simulink model "Green_Hydrogen_Model"  (R2026a)
settings: Solver=FixedStepAuto  StopTime=24*3600*365-3600  FixedStep=Ts  AbsTol=1e-3
InitFcn:
  | Ts = 3600;
values from neighbouring files (symbols this model uses):
  zstorage = 5    [initData.mat]
undefined symbols (not defined in the file or in its folder): DiscIntNeverNeededParam
libraries: fl_lib x58, nesl_utility x17, simulink x3, ee_lib x1
CloseFcn:
  | try,close(h1_ee_solar_cell),end
  | clear h1_ee_solar_cell
  | 
  | 
  | clear simlog_ee_solar_cell
  | clear logsout_ee_solar_cell
  | clear I Pmax V_Pmax idx index irradiance irradianceVec legend_info powerMat powerTable temperature temperatureVec vVec voltageTable
Description:
  | Solar Cell Power Curve
settings Model: Creator=The MathWorks, Inc.  LastModifiedBy=aayushi
settings SolverCC: InitialStep=0.1
settings DataIOCC: ExternalInput=[(0:3600:3600*24*365-3600)' irradiance]  LoadExternalInput=on  SaveFormat=StructureWithTime  InspectSignalLogs=on  SignalLoggingName=y  OutputOption=SpecifiedOutputTimes  OutputTimes=[0:0.5:60]
settings DebuggingCC: UnderspecifiedInitializationDetection=Classic
settings HardwareCC: ProdHWDeviceType=32-bit Generic
settings GRTTargetCC: CombineOutputUpdateFcns=off  GRTInterface=on
settings SimscapeCC: SimscapeNormalizeSystem=off  SimscapeNominalValues="[{\"value\":\"1\",\"unit\":\"A\"},{\"value\":\"1\",\"unit\":\"bar\"},{\"value\":\"1\",\"unit\":\"cm^2\"},{\"value\":\"1\",\"unit\":\"cm^3/s\"},{\"value\":\"1\",\"unit\":\"kJ/kg\"},{\"value\":\"1\",\"unit\":\"kW\"},{\"value\":\"1\",\"unit\":\"l\"},{\"value\":\"1\",\"unit\":\"N\"},{\"value\":\"1\",\"unit\":\"N*m\"},{\"value\":\"1\",\"unit\":\"V\"}]"  SimscapeLogType=none  SimscapeLogName=simlog_ee_solar_cell  SimscapeLogLimitData=off

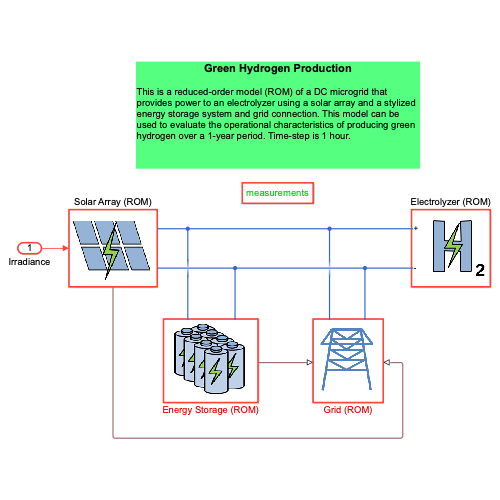
[thumbnail: Simulink's stored preview of the top-level diagram]
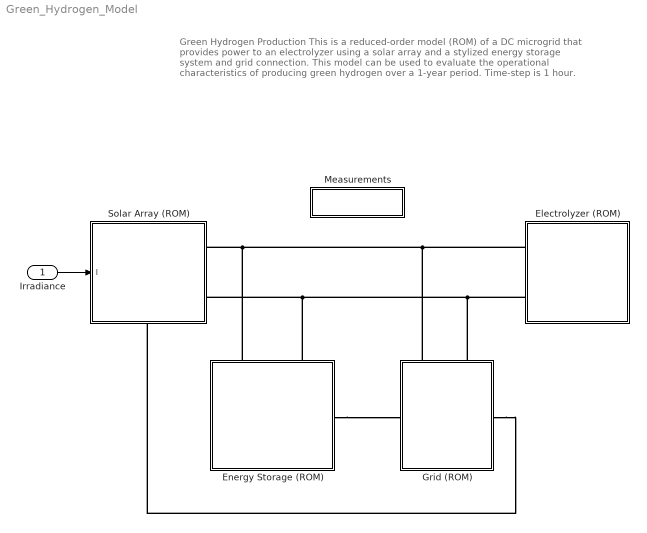
== system Green_Hydrogen_Model ==
  note: Green Hydrogen Production
      |
      | This is a reduced-order model (ROM) of a DC microgrid that provides power to an electrolyzer using a solar array and a stylized energy storage system and grid connection. This model can be used to evaluate the operational characteristics of producing green hydrogen over a 1-year period. Time-step is 1 hour.
  Irradiance : Inport  PortDimensions=1
  Electrolyzer (ROM) : Subsystem
      mask Display: image(imread('green_hydrogen.png'))
  Energy Storage (ROM) : Subsystem
      settings: PortSchema="{\"entries\":[{\"content\":{\"sides\":[{\"content\":{\"connectorIds\":[]},\"type\":\"ConnectorPlacement.EquallySpacedRectSide\",\"uuid\":\"4ce9e896-492d-4425-b4ff-f24d4b5e5863\"},{\"content\":{\"connectorIds\":[\"RConn1\"],\"side\":\"RIGHT\"},\"type\":\"ConnectorPlacement.EquallySpacedRectSide\",\"uuid\":\"930c7228-c80c-44c8-ab76-5d29522f1c4f\"},{\"content\":{\"connectorIds\":[\"LConn1\",\"LConn2\"],\"side\":\"TOP\"},\"type\":\"ConnectorPlacement.EquallySpacedRectSide\",\"uuid\":\"6c2706e8-63c7-47cf-ac96-eabca5dbf54e\"}]},\"type\":\"ConnectorPlacement.EquallySpacedConnector\",\"uuid\":\"1ee3078e-0db2-4038-8bbf-aa4f1eaec25a\"}],\"packageUris\":[\"http://schema.mathworks.com/mf0/Connector/R2020b\"],\"version\":\"1.0\"}"
      mask Display: image(imread('storage.png'))
  Grid (ROM) : Subsystem
      settings: PortSchema="{\"entries\":[{\"content\":{\"sides\":[{\"content\":{\"connectorIds\":[\"LConn1\"]},\"type\":\"ConnectorPlacement.EquallySpacedRectSide\",\"uuid\":\"4ce9e896-492d-4425-b4ff-f24d4b5e5863\"},{\"content\":{\"connectorIds\":[\"RConn1\"],\"side\":\"RIGHT\"},\"type\":\"ConnectorPlacement.EquallySpacedRectSide\",\"uuid\":\"930c7228-c80c-44c8-ab76-5d29522f1c4f\"},{\"content\":{\"connectorIds\":[\"LConn2\",\"LConn3\"],\"side\":\"TOP\"},\"type\":\"ConnectorPlacement.EquallySpacedRectSide\",\"uuid\":\"6c2706e8-63c7-47cf-ac96-eabca5dbf54e\"},{\"content\":{\"connectorIds\":[],\"side\":\"BOTTOM\"},\"type\":\"ConnectorPlacement.EquallySpacedRectSide\",\"uuid\":\"490b5229-98f3-4f3a-9ef5-f546c826e2d2\"}]},\"type\":\"ConnectorPlacement.EquallySpacedConnector\",\"uuid\":\"1ee3078e-0db2-4038-8bbf-aa4f1eaec25a\"}],\"packageUris\":[\"http://schema.mathworks.com/mf0/Connector/R2020b\"],\"version\":\"1.0\"}"
      mask Display: image(imread('grid.png'))
  Measurements : Subsystem
      mask Display: disp('measurements')
  Solar Array (ROM) : Subsystem
      settings: PortSchema="{\"entries\":[{\"content\":{\"sides\":[{\"content\":{\"connectorIds\":[\"In1\"]},\"type\":\"ConnectorPlacement.EquallySpacedRectSide\",\"uuid\":\"a867b3ed-c44d-46d3-b035-bd7f0843dcab\"},{\"content\":{\"connectorIds\":[\"RConn1\",\"RConn2\"],\"side\":\"RIGHT\"},\"type\":\"ConnectorPlacement.EquallySpacedRectSide\",\"uuid\":\"5b118fd7-24ef-441f-9afe-5591aca8fd6c\"},{\"content\":{\"connectorIds\":[],\"side\":\"TOP\"},\"type\":\"ConnectorPlacement.EquallySpacedRectSide\",\"uuid\":\"b5b5fc8b-bb18-419b-a077-b902c124e389\"},{\"content\":{\"connectorIds\":[\"RConn3\"],\"side\":\"BOTTOM\"},\"type\":\"ConnectorPlacement.EquallySpacedRectSide\",\"uuid\":\"62f7ab30-8438-4320-a8c5-25a9418176a3\"}]},\"type\":\"ConnectorPlacement.EquallySpacedConnector\",\"uuid\":\"ded5530a-2615-43e4-9f45-04d72cddf901\"}],\"packageUris\":[\"http://schema.mathworks.com/mf0/Connector/R2020b\"],\"version\":\"1.0\"}"
      mask Display: image(imread('solar.png'))
  wires:
  Irradiance/1 -> Solar Array (ROM)/1(I)
  connections:
  Electrolyzer (ROM)/LConn1 -- Solar Array (ROM)/RConn1 -- Energy Storage (ROM)/LConn1 -- Grid (ROM)/LConn2
  Electrolyzer (ROM)/LConn2 -- Solar Array (ROM)/RConn2 -- Energy Storage (ROM)/LConn2 -- Grid (ROM)/LConn3
  Grid (ROM)/RConn1 -- Solar Array (ROM)/RConn3
  Energy Storage (ROM)/RConn1 -- Grid (ROM)/LConn1

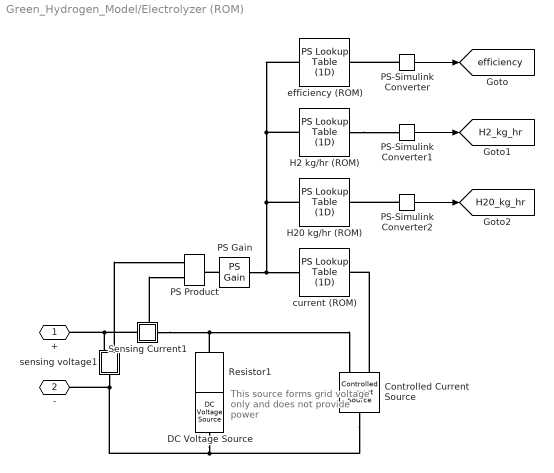
== system Green_Hydrogen_Model/Electrolyzer (ROM) ==
  note: This source forms grid voltage only and does not provide power
  Controlled Current Source : fl_lib/Electrical/Electrical Sources/Controlled Current Source
  DC Voltage Source : fl_lib/Electrical/Electrical Sources/DC Voltage Source  v0=240 V
  H2 kg/hr (ROM) : fl_lib/Physical Signals/Lookup Tables/PS Lookup Table (1D)  x=powerv  f=H2_kg_hr  interp_method=simscape.enum.interpolation.linear  extrap_method=simscape.enum.extrapolation.linear
  H20 kg/hr (ROM) : fl_lib/Physical Signals/Lookup Tables/PS Lookup Table (1D)  x=powerv  f=H20_kg_hr  interp_method=simscape.enum.interpolation.linear  extrap_method=simscape.enum.extrapolation.linear
  PS Gain : fl_lib/Physical Signals/Functions/PS Gain  gain=1 1/V/A
  PS Product : fl_lib/Physical Signals/Functions/PS Product
  PS-Simulink Converter : nesl_utility/PS-Simulink Converter  PhysicalDomain=network_engine_domain  SubClassName=ps_output  LeftPortType=input  RightPortType=output  PseudoPeriodic=off  Frequencies=[]  VectorFormat=1-D array  Unit=inherit  AffineConversion=off
  PS-Simulink Converter1 : nesl_utility/PS-Simulink Converter  PhysicalDomain=network_engine_domain  SubClassName=ps_output  LeftPortType=input  RightPortType=output  PseudoPeriodic=off  Frequencies=[]  VectorFormat=1-D array  Unit=inherit  AffineConversion=off
  PS-Simulink Converter2 : nesl_utility/PS-Simulink Converter  PhysicalDomain=network_engine_domain  SubClassName=ps_output  LeftPortType=input  RightPortType=output  PseudoPeriodic=off  Frequencies=[]  VectorFormat=1-D array  Unit=inherit  AffineConversion=off
  Resistor1 : fl_lib/Electrical/Electrical Elements/Resistor  R=5 Ohm  i_specify=off  i_priority=None  i=0 A  i_nominal_specify=off  i_nominal_value=1  i_nominal_unit=A  v_specify=on  v_priority=None  v=240 V  v_nominal_specify=off  v_nominal_value=1  v_nominal_unit=V
  Sensing Current1 : Subsystem
      settings: PortSchema="{\"entries\":[{\"content\":{\"sides\":[{\"content\":{\"connectorIds\":[\"LConn1\"]},\"type\":\"ConnectorPlacement.EquallySpacedRectSide\",\"uuid\":\"b94629f0-79a7-4e9f-9b19-2ebf3bcf4c67\"},{\"content\":{\"connectorIds\":[\"RConn1\"],\"side\":\"RIGHT\"},\"type\":\"ConnectorPlacement.EquallySpacedRectSide\",\"uuid\":\"77befbbf-81fe-4980-a27e-5f206100ddc5\"},{\"content\":{\"connectorIds\":[\"LConn2\"],\"side\":\"TOP\"},\"type\":\"ConnectorPlacement.EquallySpacedRectSide\",\"uuid\":\"ab227c1c-b66c-46e2-a5f4-7af885246fc6\"}]},\"type\":\"ConnectorPlacement.EquallySpacedConnector\",\"uuid\":\"a3cb571c-cd46-4237-8ad8-7e1205d20cc0\"}],\"packageUris\":[\"http://schema.mathworks.com/mf0/Connector/R2020b\"],\"version\":\"1.0\"}"
      mask Display: disp('i')
  current (ROM) : fl_lib/Physical Signals/Lookup Tables/PS Lookup Table (1D)  x=powerv  f=electrolyzer_current  interp_method=simscape.enum.interpolation.linear  extrap_method=simscape.enum.extrapolation.linear
  efficiency (ROM) : fl_lib/Physical Signals/Lookup Tables/PS Lookup Table (1D)  x=powerv  f=electrolyzer_efficiency  interp_method=simscape.enum.interpolation.linear  extrap_method=simscape.enum.extrapolation.linear
  sensing voltage1 : Subsystem
      mask Display: disp('v')
  + : PMIOPort  Side=Left
  - : PMIOPort  Port=2  Side=Left
  tag scope: H20_kg_hr=global, H2_kg_hr=global, efficiency=global
  wires:
  PS-Simulink Converter/1 -> [efficiency]
  PS-Simulink Converter1/1 -> [H2_kg_hr]
  PS-Simulink Converter2/1 -> [H20_kg_hr]
  connections:
  sensing voltage1/LConn1 -- Sensing Current1/LConn1 -- +/RConn1
  sensing voltage1/RConn1 -- DC Voltage Source/RConn1 -- Controlled Current Source/LConn1 -- -/RConn1
  Sensing Current1/LConn2 -- PS Product/LConn2
  sensing voltage1/LConn2 -- PS Product/LConn1
  PS Gain/LConn1 -- PS Product/RConn1
  Controlled Current Source/RConn1 -- current (ROM)/RConn1
  Sensing Current1/RConn1 -- Resistor1/LConn1 -- Controlled Current Source/RConn2
  DC Voltage Source/LConn1 -- Resistor1/RConn1
  PS-Simulink Converter/LConn1 -- efficiency (ROM)/RConn1
  PS-Simulink Converter2/LConn1 -- H20 kg/hr (ROM)/RConn1
  H2 kg/hr (ROM)/RConn1 -- PS-Simulink Converter1/LConn1
  PS Gain/RConn1 -- current (ROM)/LConn1 -- H20 kg/hr (ROM)/LConn1 -- efficiency (ROM)/LConn1 -- H2 kg/hr (ROM)/LConn1

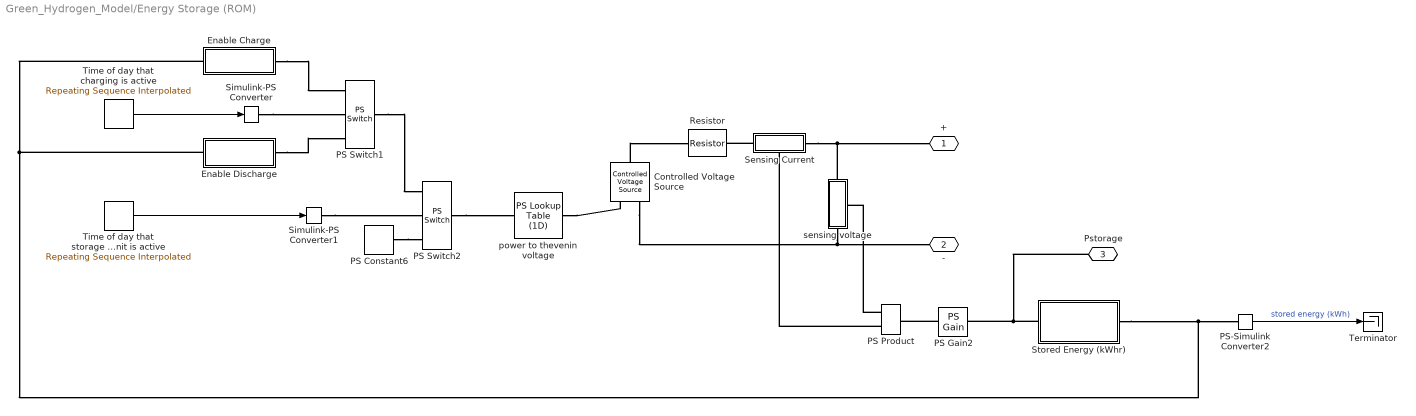
== system Green_Hydrogen_Model/Energy Storage (ROM) ==
  Controlled Voltage Source : fl_lib/Electrical/Electrical Sources/Controlled Voltage Source
  Enable Charge : Subsystem
  Enable Discharge : Subsystem
  PS Constant6 : fl_lib/Physical Signals/Sources/PS Constant  constant=0
  PS Gain2 : fl_lib/Physical Signals/Functions/PS Gain  gain=1 1/V/A
  PS Product : fl_lib/Physical Signals/Functions/PS Product
  PS Switch1 : fl_lib/Physical Signals/Nonlinear Operators/PS Switch  Threshold=0.99  ZeroCross=true
  PS Switch2 : fl_lib/Physical Signals/Nonlinear Operators/PS Switch  Threshold=0.99  ZeroCross=true
  PS-Simulink Converter2 : nesl_utility/PS-Simulink Converter  PhysicalDomain=network_engine_domain  SubClassName=ps_output  LeftPortType=input  RightPortType=output  PseudoPeriodic=off  Frequencies=[]  VectorFormat=1-D array  Unit=inherit  AffineConversion=off
  Resistor : fl_lib/Electrical/Electrical Elements/Resistor  R=zstorage Ohm  i_specify=off  i_priority=None  i=0 A  i_nominal_specify=off  i_nominal_value=1  i_nominal_unit=A  v_specify=off  v_priority=None  v=0 V  v_nominal_specify=off  v_nominal_value=1  v_nominal_unit=V
  Sensing Current : Subsystem
      settings: PortSchema="{\"entries\":[{\"content\":{\"sides\":[{\"content\":{\"connectorIds\":[\"LConn1\"]},\"type\":\"ConnectorPlacement.EquallySpacedRectSide\",\"uuid\":\"c99cf1a8-fc4f-439f-81a5-065ef56794a1\"},{\"content\":{\"connectorIds\":[\"RConn1\"],\"side\":\"RIGHT\"},\"type\":\"ConnectorPlacement.EquallySpacedRectSide\",\"uuid\":\"2fde9b7a-e051-4c9e-865a-56b031831294\"},{\"content\":{\"connectorIds\":[],\"side\":\"TOP\"},\"type\":\"ConnectorPlacement.EquallySpacedRectSide\",\"uuid\":\"fbc77884-485b-4fd8-805c-e7a3dc707aba\"},{\"content\":{\"connectorIds\":[\"RConn2\"],\"side\":\"BOTTOM\"},\"type\":\"ConnectorPlacement.EquallySpacedRectSide\",\"uuid\":\"a7518d99-1e9b-4c67-b1d7-16fc35a4cea4\"}]},\"type\":\"ConnectorPlacement.EquallySpacedConnector\",\"uuid\":\"18321e03-afa8-4af1-9a2f-bf6413052394\"}],\"packageUris\":[\"http://schema.mathworks.com/mf0/Connector/R2020b\"],\"version\":\"1.0\"}"
      mask Display: disp('i')
  Simulink-PS Converter : nesl_utility/Simulink-PS Converter  PhysicalDomain=network_engine_domain  SubClassName=ps_input  LeftPortType=input  RightPortType=output  PseudoPeriodic=off  Frequencies=[]  NoiseDistribution=none  NoiseParameters=[]  Unit=1  AffineConversion=off  FilteringAndDerivatives=provide  SimscapeFilterOrder=1  InputFilterTimeConstant=0.001  UdotUserProvided=0
  Simulink-PS Converter1 : nesl_utility/Simulink-PS Converter  PhysicalDomain=network_engine_domain  SubClassName=ps_input  LeftPortType=input  RightPortType=output  PseudoPeriodic=off  Frequencies=[]  NoiseDistribution=none  NoiseParameters=[]  Unit=1  AffineConversion=off  FilteringAndDerivatives=provide  SimscapeFilterOrder=1  InputFilterTimeConstant=0.001  UdotUserProvided=0
  Stored Energy (kWhr) : Subsystem
  Terminator : Terminator
  Time of day that charging is active : simulink/Sources/Repeating Sequence Interpolated  OutValues=[0 0 1 1 0 0]  TimeValues=[0 8*3600-Ts 8*3600 14*3600-Ts 14*3600 24*3600-Ts]  LookUpMeth=Interpolation-Use End Values  tsamp=Ts  OutMin=[]  OutMax=[]  OutDataTypeStr=double  OutputDataTypeScalingMode=double  OutDataType=fixdt(0,8)  OutScaling=2^-10
  Time of day that storage unit is active : simulink/Sources/Repeating Sequence Interpolated  OutValues=[0 0 1 1 0 0 1 1]  TimeValues=[0 6*3600-Ts 6*3600 12*3600-Ts 12*3600 20*3600-Ts 20*3600 24*3600-Ts]  LookUpMeth=Interpolation-Use End Values  tsamp=Ts  OutMin=[]  OutMax=[]  OutDataTypeStr=double  OutputDataTypeScalingMode=double  OutDataType=fixdt(0,8)  OutScaling=2^-10
  power to thevenin voltage : fl_lib/Physical Signals/Lookup Tables/PS Lookup Table (1D)  x=pstorage  f=vstorage  interp_method=simscape.enum.interpolation.linear  extrap_method=simscape.enum.extrapolation.linear
  sensing voltage : Subsystem
      settings: PortSchema="{\"entries\":[{\"content\":{\"sides\":[{\"content\":{\"connectorIds\":[\"LConn1\"]},\"type\":\"ConnectorPlacement.EquallySpacedRectSide\",\"uuid\":\"174cc4c7-8d7f-48d2-a7e2-2f35130ccdcd\"},{\"content\":{\"connectorIds\":[\"RConn1\"],\"side\":\"RIGHT\"},\"type\":\"ConnectorPlacement.EquallySpacedRectSide\",\"uuid\":\"9e60102e-41cf-47d2-a399-aa8583a1bfd5\"},{\"content\":{\"connectorIds\":[],\"side\":\"TOP\"},\"type\":\"ConnectorPlacement.EquallySpacedRectSide\",\"uuid\":\"1bf2b277-65ab-4966-a80f-8100630a083b\"},{\"content\":{\"connectorIds\":[\"RConn2\"],\"side\":\"BOTTOM\"},\"type\":\"ConnectorPlacement.EquallySpacedRectSide\",\"uuid\":\"735a8926-423a-42f4-bd5d-475d3049eafb\"}]},\"type\":\"ConnectorPlacement.EquallySpacedConnector\",\"uuid\":\"1a25aba2-97b0-44d7-b65c-a2aa0aac9e6e\"}],\"packageUris\":[\"http://schema.mathworks.com/mf0/Connector/R2020b\"],\"version\":\"1.0\"}"
      mask Display: disp('v')
  + : PMIOPort  Side=Left
  - : PMIOPort  Port=2  Side=Left
  Pstorage : PMIOPort  Port=3  Side=Right
  wires:
  PS-Simulink Converter2/1 -> Terminator/1  "stored energy (kWh)"
  Time of day that charging is active/1 -> Simulink-PS Converter/1
  Time of day that storage unit is active/1 -> Simulink-PS Converter1/1
  connections:
  Controlled Voltage Source/LConn1 -- Resistor/RConn1
  Controlled Voltage Source/RConn2 -- sensing voltage/RConn1 -- -/RConn1
  Sensing Current/LConn1 -- Resistor/LConn1
  Sensing Current/RConn1 -- sensing voltage/LConn1 -- +/RConn1
  PS Product/LConn1 -- sensing voltage/RConn2
  PS Product/LConn2 -- Sensing Current/RConn2
  PS Gain2/LConn1 -- PS Product/RConn1
  power to thevenin voltage/RConn1 -- Controlled Voltage Source/RConn1
  PS Switch1/RConn1 -- PS Switch2/LConn1
  PS Constant6/RConn1 -- PS Switch2/LConn3
  PS Switch2/RConn1 -- power to thevenin voltage/LConn1
  Simulink-PS Converter/RConn1 -- PS Switch1/LConn2
  Simulink-PS Converter1/RConn1 -- PS Switch2/LConn2
  Pstorage/RConn1 -- Stored Energy (kWhr)/LConn1 -- PS Gain2/RConn1
  Enable Discharge/RConn1 -- PS Switch1/LConn3
  Stored Energy (kWhr)/RConn1 -- Enable Charge/LConn1 -- Enable Discharge/LConn1 -- PS-Simulink Converter2/LConn1
  Enable Charge/RConn1 -- PS Switch1/LConn1

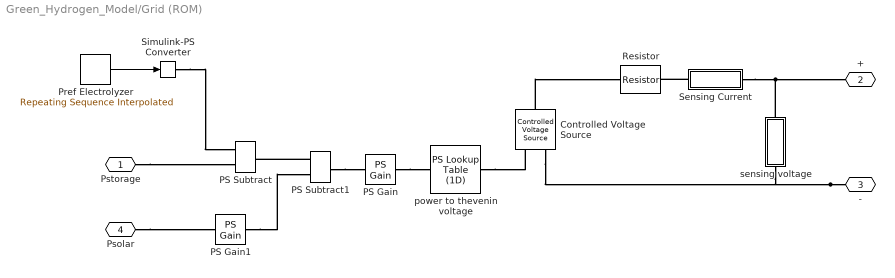
== system Green_Hydrogen_Model/Grid (ROM) ==
  Controlled Voltage Source : fl_lib/Electrical/Electrical Sources/Controlled Voltage Source
  PS Gain : fl_lib/Physical Signals/Functions/PS Gain  gain=1
  PS Gain1 : fl_lib/Physical Signals/Functions/PS Gain  gain=1 1/V/A
  PS Subtract : fl_lib/Physical Signals/Functions/PS Subtract
  PS Subtract1 : fl_lib/Physical Signals/Functions/PS Subtract
  Pref Electrolyzer : simulink/Sources/Repeating Sequence Interpolated  OutValues=[0.01 0.01 1 1 1 1]*150e3  TimeValues=[0 8*3600-Ts 8*3600 20*3600-Ts 20*3600 24*3600-Ts]  LookUpMeth=Interpolation-Use End Values  tsamp=Ts  OutMin=[]  OutMax=[]  OutDataTypeStr=double  OutputDataTypeScalingMode=double  OutDataType=fixdt(0,8)  OutScaling=2^-10
  Resistor : fl_lib/Electrical/Electrical Elements/Resistor  R=zstorage Ohm  i_specify=off  i_priority=None  i=0 A  i_nominal_specify=off  i_nominal_value=1  i_nominal_unit=A  v_specify=off  v_priority=None  v=0 V  v_nominal_specify=off  v_nominal_value=1  v_nominal_unit=V
  Sensing Current : Subsystem
      mask Display: disp('i')
  Simulink-PS Converter : nesl_utility/Simulink-PS Converter  PhysicalDomain=network_engine_domain  SubClassName=ps_input  LeftPortType=input  RightPortType=output  PseudoPeriodic=off  Frequencies=[]  NoiseDistribution=none  NoiseParameters=[]  Unit=1  AffineConversion=off  FilteringAndDerivatives=provide  SimscapeFilterOrder=1  InputFilterTimeConstant=0.001  UdotUserProvided=0
  power to thevenin voltage : fl_lib/Physical Signals/Lookup Tables/PS Lookup Table (1D)  x=pstorage  f=vstorage  interp_method=simscape.enum.interpolation.linear  extrap_method=simscape.enum.extrapolation.linear
  sensing voltage : Subsystem
      mask Display: disp('v')
  Pstorage : PMIOPort  Side=Left
  + : PMIOPort  Port=2  Side=Left
  - : PMIOPort  Port=3  Side=Left
  Psolar : PMIOPort  Port=4  Side=Right
  wires:
  Pref Electrolyzer/1 -> Simulink-PS Converter/1
  connections:
  PS Gain/RConn1 -- power to thevenin voltage/LConn1
  sensing voltage/LConn1 -- Sensing Current/RConn1 -- +/RConn1
  Sensing Current/LConn1 -- Resistor/LConn1
  power to thevenin voltage/RConn1 -- Controlled Voltage Source/RConn1
  -/RConn1 -- Controlled Voltage Source/RConn2 -- sensing voltage/RConn1
  Controlled Voltage Source/LConn1 -- Resistor/RConn1
  Pstorage/RConn1 -- PS Subtract/LConn2
  PS Subtract1/LConn1 -- PS Subtract/RConn1
  PS Gain1/RConn1 -- PS Subtract1/LConn2
  PS Subtract1/RConn1 -- PS Gain/LConn1
  Psolar/RConn1 -- PS Gain1/LConn1
  Simulink-PS Converter/RConn1 -- PS Subtract/LConn1

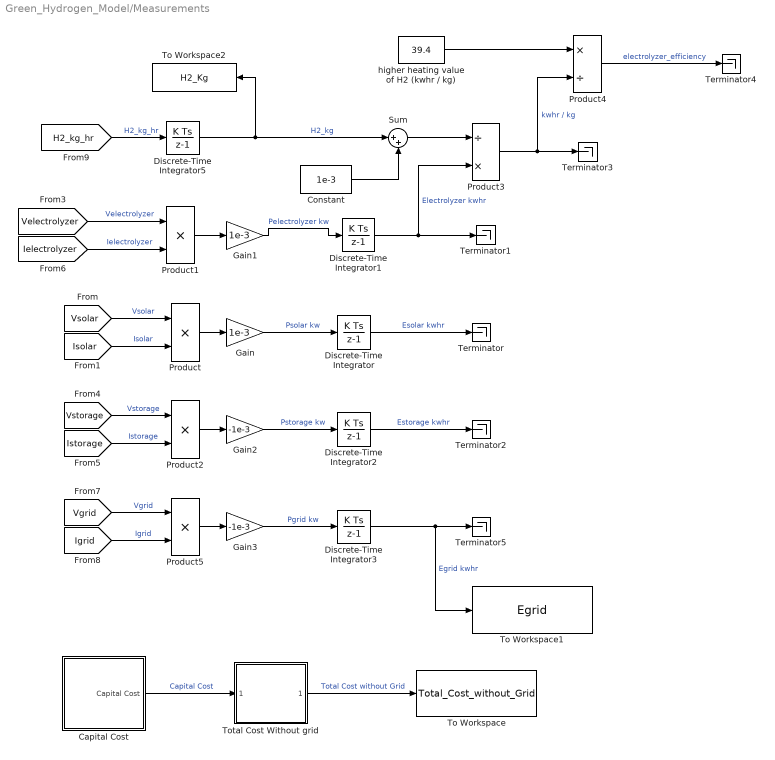
== system Green_Hydrogen_Model/Measurements ==
  Capital Cost : Subsystem
      mask Display: image('$imagefile'); % Use "Edit Image" on toolstrip to change.
  Constant : Constant  Value=1e-3  SampleTime=Ts
  Discrete-Time Integrator : DiscreteIntegrator  gainval=1/3600  SampleTime=-1  ICPrevOutput=DiscIntNeverNeededParam  ICPrevScaledInput=DiscIntNeverNeededParam
  Discrete-Time Integrator1 : DiscreteIntegrator  gainval=1/3600  SampleTime=-1  ICPrevOutput=DiscIntNeverNeededParam  ICPrevScaledInput=DiscIntNeverNeededParam
  Discrete-Time Integrator2 : DiscreteIntegrator  gainval=1/3600  InitialCondition=1000  SampleTime=-1  ICPrevOutput=DiscIntNeverNeededParam  ICPrevScaledInput=DiscIntNeverNeededParam
  Discrete-Time Integrator3 : DiscreteIntegrator  gainval=1/3600  InitialCondition=1000  SampleTime=-1  ICPrevOutput=DiscIntNeverNeededParam  ICPrevScaledInput=DiscIntNeverNeededParam
  Discrete-Time Integrator5 : DiscreteIntegrator  gainval=1/3600  SampleTime=-1  ICPrevOutput=DiscIntNeverNeededParam  ICPrevScaledInput=DiscIntNeverNeededParam
  Gain : Gain  Gain=1e-3
  Gain1 : Gain  Gain=1e-3
  Gain2 : Gain  Gain=-1e-3
  Gain3 : Gain  Gain=-1e-3
  Product{,1..2,5} (4 alike) : Product
  Product3 : Product  Inputs=/*
  Product4 : Product  Inputs=*/
  Sum : Sum  Inputs=|++
  Terminator{,1..5} (6 alike) : Terminator
  To Workspace : ToWorkspace  VariableName=Total_Cost_without_Grid  SaveFormat=Structure With Time  SampleTime=-1
  To Workspace1 : ToWorkspace  VariableName=Egrid  SaveFormat=Structure With Time  SampleTime=-1
  To Workspace2 : ToWorkspace  VariableName=H2_Kg  SaveFormat=Structure With Time  SampleTime=-1
  Total Cost Without grid : Subsystem
      mask Display: image('$imagefile'); % Use "Edit Image" on toolstrip to change.
  higher heating value of H2 (kwhr / kg) : Constant  Value=39.4  SampleTime=Ts
  wires:
  Constant/1 -> Sum/2
  [Istorage] -> Product2/2  "Istorage"
  Product4/1 -> Terminator4/1  "electrolyzer_efficiency"
  Discrete-Time Integrator3/1 -> To Workspace1/1, Terminator5/1  "Egrid kwhr"
  [Vstorage] -> Product2/1  "Vstorage"
  [Isolar] -> Product/2  "Isolar"
  [Vgrid] -> Product5/1  "Vgrid"
  Discrete-Time Integrator/1 -> Terminator/1  "Esolar kwhr"
  Gain1/1 -> Discrete-Time Integrator1/1  "Pelectrolyzer kw"
  higher heating value of H2 (kwhr / kg)/1 -> Product4/1
  Product3/1 -> Product4/2, Terminator3/1  "kwhr / kg"
  [H2_kg_hr] -> Discrete-Time Integrator5/1  "H2_kg_hr"
  [Vsolar] -> Product/1  "Vsolar"
  Product2/1 -> Gain2/1
  Sum/1 -> Product3/1
  Product5/1 -> Gain3/1
  Discrete-Time Integrator1/1 -> Product3/2, Terminator1/1  "Electrolyzer kwhr"
  [Velectrolyzer] -> Product1/1  "Velectrolyzer"
  Gain/1 -> Discrete-Time Integrator/1  "Psolar kw"
  Product/1 -> Gain/1
  Gain2/1 -> Discrete-Time Integrator2/1  "Pstorage kw"
  [Ielectrolyzer] -> Product1/2  "Ielectrolyzer"
  Discrete-Time Integrator5/1 -> To Workspace2/1, Sum/1  "H2_kg"
  Product1/1 -> Gain1/1
  [Igrid] -> Product5/2  "Igrid"
  Discrete-Time Integrator2/1 -> Terminator2/1  "Estorage kwhr"
  Gain3/1 -> Discrete-Time Integrator3/1  "Pgrid kw"
  Total Cost Without grid/1(Total Cost without Grid) -> To Workspace/1  "Total Cost without Grid"
  Capital Cost/1(Capital Cost) -> Total Cost Without grid/1(Capital Cost)  "Capital Cost"

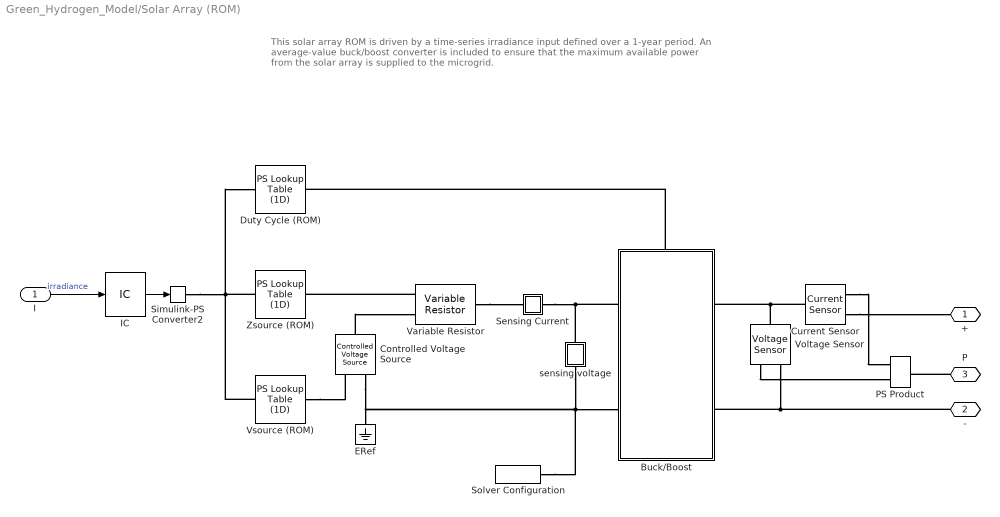
== system Green_Hydrogen_Model/Solar Array (ROM) ==
  note: This solar array ROM is driven by a time-series irradiance input defined over a 1-year period. An average-value buck/boost converter is included to ensure that the maximum available power from the solar array is supplied to the microgrid.
  I : Inport
  Buck/Boost : Subsystem
      settings: PortSchema="{\"entries\":[{\"content\":{\"sides\":[{\"content\":{\"connectorIds\":[\"LConn1\",\"LConn2\"]},\"type\":\"ConnectorPlacement.EquallySpacedRectSide\",\"uuid\":\"59b30d2c-2033-428e-a6b3-b4d8d7ac74c4\"},{\"content\":{\"connectorIds\":[\"RConn1\",\"RConn2\"],\"side\":\"RIGHT\"},\"type\":\"ConnectorPlacement.EquallySpacedRectSide\",\"uuid\":\"63b32dc2-a1f5-4b5e-a815-fc0940ceb55f\"},{\"content\":{\"connectorIds\":[\"LConn3\"],\"side\":\"TOP\"},\"type\":\"ConnectorPlacement.EquallySpacedRectSide\",\"uuid\":\"119f0c3e-2c24-4ca2-93c7-23abc773056f\"}]},\"type\":\"ConnectorPlacement.EquallySpacedConnector\",\"uuid\":\"ce7de34e-cf8c-4407-a47e-2188a402b483\"}],\"packageUris\":[\"http://schema.mathworks.com/mf0/Connector/R2020b\"],\"version\":\"1.0\"}"
  Controlled Voltage Source : fl_lib/Electrical/Electrical Sources/Controlled Voltage Source
  Current Sensor : fl_lib/Electrical/Electrical Sensors/Current Sensor
  Duty Cycle (ROM) : fl_lib/Physical Signals/Lookup Tables/PS Lookup Table (1D)  x=irrv  f=duty_cycle_ROM  interp_method=simscape.enum.interpolation.linear  extrap_method=simscape.enum.extrapolation.linear
  ERef : fl_lib/Electrical/Electrical Elements/Electrical Reference
  IC : InitialCondition  Value=10000
  PS Product : fl_lib/Physical Signals/Functions/PS Product
  Sensing Current : Subsystem
      mask Display: disp('i')
  Simulink-PS Converter2 : nesl_utility/Simulink-PS Converter  PhysicalDomain=network_engine_domain  SubClassName=ps_input  LeftPortType=input  RightPortType=output  PseudoPeriodic=off  Frequencies=[]  NoiseDistribution=none  NoiseParameters=[]  Unit=1  AffineConversion=off  FilteringAndDerivatives=provide  SimscapeFilterOrder=1  InputFilterTimeConstant=0.001  UdotUserProvided=0
  Solver Configuration : nesl_utility/Solver Configuration  PhysicalDomain=network_engine_domain  SubClassName=solver  LeftPortType=input  RightPortType=generic  Tones=[]  Harmonics=[]  SimulateNoise=off  Profile=off  UseLocalSampling=off  EnableSwitchedLinearOptims=on  FrequencyDomain=off  UseCCode=off  RelTol=0.001  AbsTol=1e-06  MinStep=1e-09  ToWorkspace=off  RevertToSquareIcSolve=off  NumHomotopyIterations=100  PhasorMode=off  PhasorModeNumHarmonics=1  ConsistencySolver=NEWTON_FTOL  CanonicalOrdering=UNORDERED  OptimizeIntermediates=UNOPTIMIZED  IndexReductionMethod=DerivativeReplacement  DoDC=on  ResidualTolerance=1e-9  ConsistencyTolSource=GLOBAL  ConsistencyAbsTol=0.001  ConsistencyRelTol=0.001  ConsistencyTolFactor=0.001  UseLocalSolver=on  LocalSolverChoice=NE_BACKWARD_EULER_ADVANCER  ResolveIndetEquations=on  FunctionEvalNumThread=1  LocalSolverSampleTime=Ts  DoFixedCost=on  MaxNonlinIter=4  MaxModeIter=2  ComputeImpulses=off  ImpulseIterations=2  LinearAlgebra=Sparse  LinearAlgebraNumThread=0  EquationFormulation=NE_TIME_EF  DelaysMemoryBudget=1024  AutomaticFiltering=off  FilteringTimeConstant=0.001  PartitionStorageMethod=AS_NEEDED  PartitionMemoryBudget=1024  PartitionMethod=FAST  MultibodyUseLocalSolver=off  MultibodyLocalSolverChoice=ODE1  MultibodyLocalSolverSampleTime=0.001
  Variable Resistor : fl_lib/Electrical/Electrical Elements/Variable Resistor  Rmin=0 Ohm  thermalEnable=false  thermal_mass=1 J/K  i_specify=off  i_priority=None  i=0 A  i_nominal_specify=off  i_nominal_value=1  i_nominal_unit=A  v_specify=off  v_priority=None  v=0 V  v_nominal_specify=off  v_nominal_value=1  v_nominal_unit=V  T_specify=off  T_priority=None  T=300 K  T_nominal_specify=off  T_nominal_value=1  T_nominal_unit=K
  Voltage Sensor : fl_lib/Electrical/Electrical Sensors/Voltage Sensor
  Vsource (ROM) : fl_lib/Physical Signals/Lookup Tables/PS Lookup Table (1D)  x=irrv  f=vsource_ROM  interp_method=simscape.enum.interpolation.linear  extrap_method=simscape.enum.extrapolation.linear
  Zsource (ROM) : fl_lib/Physical Signals/Lookup Tables/PS Lookup Table (1D)  x=irrv  f=zsource_ROM  interp_method=simscape.enum.interpolation.linear  extrap_method=simscape.enum.extrapolation.linear
  sensing voltage : Subsystem
      mask Display: disp('v')
  + : PMIOPort  Side=Right
  - : PMIOPort  Port=2  Side=Right
  P : PMIOPort  Port=3  Side=Right
  wires:
  I/1 -> IC/1  "irradiance"
  IC/1 -> Simulink-PS Converter2/1
  connections:
  Variable Resistor/RConn1 -- Sensing Current/LConn1
  Vsource (ROM)/RConn1 -- Controlled Voltage Source/RConn1
  sensing voltage/RConn1 -- Solver Configuration/RConn1 -- Buck/Boost/LConn2 -- Controlled Voltage Source/RConn2 -- ERef/LConn1
  sensing voltage/LConn1 -- Sensing Current/RConn1 -- Buck/Boost/LConn1
  Controlled Voltage Source/LConn1 -- Variable Resistor/LConn2
  Voltage Sensor/LConn1 -- Current Sensor/LConn1 -- Buck/Boost/RConn1
  Voltage Sensor/RConn2 -- -/RConn1 -- Buck/Boost/RConn2
  Current Sensor/RConn2 -- +/RConn1
  Current Sensor/RConn1 -- PS Product/LConn1
  Voltage Sensor/RConn1 -- PS Product/LConn2
  P/RConn1 -- PS Product/RConn1
  Simulink-PS Converter2/RConn1 -- Duty Cycle (ROM)/LConn1 -- Vsource (ROM)/LConn1 -- Zsource (ROM)/LConn1
  Buck/Boost/LConn3 -- Duty Cycle (ROM)/RConn1
  Variable Resistor/LConn1 -- Zsource (ROM)/RConn1

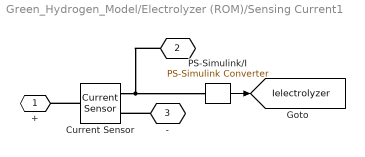
== system Green_Hydrogen_Model/Electrolyzer (ROM)/Sensing Current1 ==
  Current Sensor : fl_lib/Electrical/Electrical Sensors/Current Sensor
  PS-Simulink/I : nesl_utility/PS-Simulink Converter  PhysicalDomain=network_engine_domain  SubClassName=ps_output  LeftPortType=input  RightPortType=output  PseudoPeriodic=off  Frequencies=[]  VectorFormat=1-D array  Unit=1  AffineConversion=off
  + : PMIOPort  Side=Left
  " " : PMIOPort  Port=2  Side=Left
  - : PMIOPort  Port=3  Side=Right
  tag scope: Ielectrolyzer=global
  wires:
  PS-Simulink/I/1 -> [Ielectrolyzer]
  connections:
  -/RConn1 -- Current Sensor/RConn2
  Current Sensor/LConn1 -- +/RConn1
  Current Sensor/RConn1 -- " "/RConn1 -- PS-Simulink/I/LConn1

== system Green_Hydrogen_Model/Electrolyzer (ROM)/sensing voltage1 ==
  PS-Simulink Converter : nesl_utility/PS-Simulink Converter  PhysicalDomain=network_engine_domain  SubClassName=ps_output  LeftPortType=input  RightPortType=output  PseudoPeriodic=off  Frequencies=[]  VectorFormat=1-D array  Unit=inherit  AffineConversion=off
  Voltage Sensor : fl_lib/Electrical/Electrical Sensors/Voltage Sensor
  + : PMIOPort  Side=Left
  - : PMIOPort  Port=2  Side=Right
  " " : PMIOPort  Port=3  Side=Left
  tag scope: Velectrolyzer=global
  wires:
  PS-Simulink Converter/1 -> [Velectrolyzer]
  connections:
  Voltage Sensor/LConn1 -- +/RConn1
  Voltage Sensor/RConn2 -- -/RConn1
  Voltage Sensor/RConn1 -- " "/RConn1 -- PS-Simulink Converter/LConn1

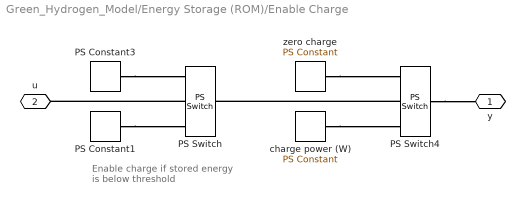
== system Green_Hydrogen_Model/Energy Storage (ROM)/Enable Charge ==
  note: Enable charge if stored energy is below threshold
  PS Constant1 : fl_lib/Physical Signals/Sources/PS Constant  constant=0
  PS Constant3 : fl_lib/Physical Signals/Sources/PS Constant  constant=1
  PS Switch : fl_lib/Physical Signals/Nonlinear Operators/PS Switch  Threshold=999  ZeroCross=true
  PS Switch4 : fl_lib/Physical Signals/Nonlinear Operators/PS Switch  Threshold=0.99  ZeroCross=true
  charge power (W) : fl_lib/Physical Signals/Sources/PS Constant  constant=-125.625e3
  zero charge : fl_lib/Physical Signals/Sources/PS Constant  constant=0
  y : PMIOPort  Side=Right
  u : PMIOPort  Port=2  Side=Left
  connections:
  zero charge/RConn1 -- PS Switch4/LConn1
  charge power (W)/RConn1 -- PS Switch4/LConn3
  PS Constant1/RConn1 -- PS Switch/LConn3
  PS Constant3/RConn1 -- PS Switch/LConn1
  PS Switch4/LConn2 -- PS Switch/RConn1
  PS Switch/LConn2 -- u/RConn1
  PS Switch4/RConn1 -- y/RConn1

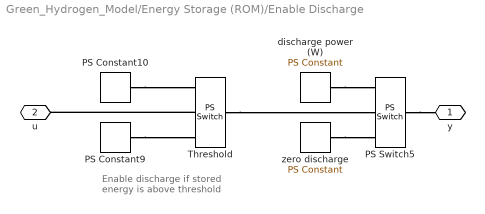
== system Green_Hydrogen_Model/Energy Storage (ROM)/Enable Discharge ==
  note: Enable discharge if stored energy is above threshold
  PS Constant10 : fl_lib/Physical Signals/Sources/PS Constant  constant=1
  PS Constant9 : fl_lib/Physical Signals/Sources/PS Constant  constant=0
  PS Switch5 : fl_lib/Physical Signals/Nonlinear Operators/PS Switch  Threshold=0.99  ZeroCross=true
  Threshold : fl_lib/Physical Signals/Nonlinear Operators/PS Switch  Threshold=50  ZeroCross=true
  discharge power (W) : fl_lib/Physical Signals/Sources/PS Constant  constant=187.5e3
  zero discharge : fl_lib/Physical Signals/Sources/PS Constant  constant=0
  y : PMIOPort  Side=Right
  u : PMIOPort  Port=2  Side=Left
  connections:
  zero discharge/RConn1 -- PS Switch5/LConn3
  Threshold/LConn2 -- u/RConn1
  PS Constant10/RConn1 -- Threshold/LConn1
  Threshold/RConn1 -- PS Switch5/LConn2
  PS Constant9/RConn1 -- Threshold/LConn3
  discharge power (W)/RConn1 -- PS Switch5/LConn1
  PS Switch5/RConn1 -- y/RConn1

== system Green_Hydrogen_Model/Energy Storage (ROM)/Sensing Current ==
  Current Sensor : fl_lib/Electrical/Electrical Sensors/Current Sensor
  PS-Simulink/I : nesl_utility/PS-Simulink Converter  PhysicalDomain=network_engine_domain  SubClassName=ps_output  LeftPortType=input  RightPortType=output  PseudoPeriodic=off  Frequencies=[]  VectorFormat=1-D array  Unit=1  AffineConversion=off
  + : PMIOPort  Side=Left
  - : PMIOPort  Port=2  Side=Right
  I : PMIOPort  Port=3  Side=Right
  tag scope: Istorage=global
  wires:
  PS-Simulink/I/1 -> [Istorage]
  connections:
  Current Sensor/RConn1 -- I/RConn1 -- PS-Simulink/I/LConn1
  Current Sensor/LConn1 -- +/RConn1
  -/RConn1 -- Current Sensor/RConn2

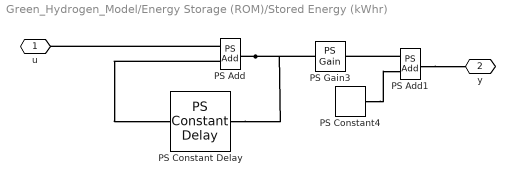
== system Green_Hydrogen_Model/Energy Storage (ROM)/Stored Energy (kWhr) ==
  PS Add : fl_lib/Physical Signals/Functions/PS Add
  PS Add1 : fl_lib/Physical Signals/Functions/PS Add
  PS Constant Delay : fl_lib/Physical Signals/Delays/PS Constant Delay  InputHistory=0  DelayTime=Ts s
  PS Constant4 : fl_lib/Physical Signals/Sources/PS Constant  constant=1000
  PS Gain3 : fl_lib/Physical Signals/Functions/PS Gain  gain=-1e-3*Ts/3600
  u : PMIOPort  Side=Left
  y : PMIOPort  Port=2  Side=Right
  connections:
  PS Add/RConn1 -- PS Gain3/LConn1 -- PS Constant Delay/LConn1
  PS Add/LConn2 -- PS Constant Delay/RConn1
  PS Add1/LConn1 -- PS Gain3/RConn1
  PS Add1/RConn1 -- y/RConn1
  PS Constant4/RConn1 -- PS Add1/LConn2
  PS Add/LConn1 -- u/RConn1

== system Green_Hydrogen_Model/Energy Storage (ROM)/sensing voltage ==
  PS-Simulink Converter : nesl_utility/PS-Simulink Converter  PhysicalDomain=network_engine_domain  SubClassName=ps_output  LeftPortType=input  RightPortType=output  PseudoPeriodic=off  Frequencies=[]  VectorFormat=1-D array  Unit=inherit  AffineConversion=off
  Voltage Sensor : fl_lib/Electrical/Electrical Sensors/Voltage Sensor
  + : PMIOPort  Side=Left
  - : PMIOPort  Port=2  Side=Right
  V : PMIOPort  Port=3  Side=Right
  tag scope: Vstorage=global
  wires:
  PS-Simulink Converter/1 -> [Vstorage]
  connections:
  Voltage Sensor/RConn1 -- PS-Simulink Converter/LConn1 -- V/RConn1
  Voltage Sensor/RConn2 -- -/RConn1
  Voltage Sensor/LConn1 -- +/RConn1

== system Green_Hydrogen_Model/Grid (ROM)/Sensing Current ==
  Current Sensor : fl_lib/Electrical/Electrical Sensors/Current Sensor
  PS-Simulink/I : nesl_utility/PS-Simulink Converter  PhysicalDomain=network_engine_domain  SubClassName=ps_output  LeftPortType=input  RightPortType=output  PseudoPeriodic=off  Frequencies=[]  VectorFormat=1-D array  Unit=1  AffineConversion=off
  + : PMIOPort  Side=Left
  - : PMIOPort  Port=2  Side=Right
  tag scope: Igrid=global
  wires:
  PS-Simulink/I/1 -> [Igrid]
  connections:
  -/RConn1 -- Current Sensor/RConn2
  Current Sensor/LConn1 -- +/RConn1
  Current Sensor/RConn1 -- PS-Simulink/I/LConn1

== system Green_Hydrogen_Model/Grid (ROM)/sensing voltage ==
  PS-Simulink Converter : nesl_utility/PS-Simulink Converter  PhysicalDomain=network_engine_domain  SubClassName=ps_output  LeftPortType=input  RightPortType=output  PseudoPeriodic=off  Frequencies=[]  VectorFormat=1-D array  Unit=inherit  AffineConversion=off
  Voltage Sensor : fl_lib/Electrical/Electrical Sensors/Voltage Sensor
  + : PMIOPort  Side=Left
  - : PMIOPort  Port=2  Side=Right
  tag scope: Vgrid=global
  wires:
  PS-Simulink Converter/1 -> [Vgrid]
  connections:
  Voltage Sensor/LConn1 -- +/RConn1
  Voltage Sensor/RConn2 -- -/RConn1
  Voltage Sensor/RConn1 -- PS-Simulink Converter/LConn1

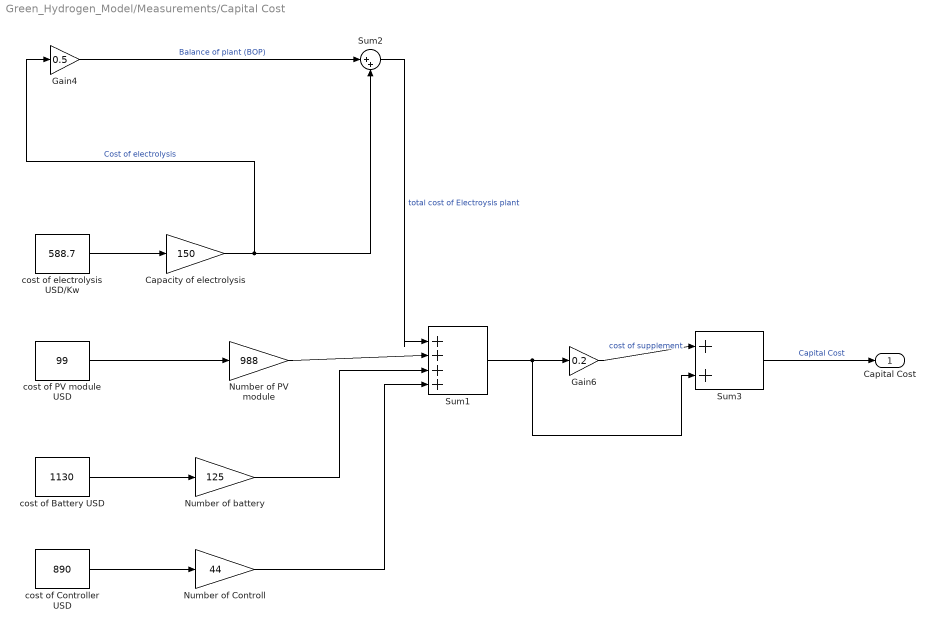
== system Green_Hydrogen_Model/Measurements/Capital Cost ==
  Capacity of electrolysis : Gain  Gain=150
  Gain4 : Gain  Gain=0.5
  Gain6 : Gain  Gain=0.2
  Number of Controll : Gain  Gain=44
  Number of PV module : Gain  Gain=988
  "Number of battery " : Gain  Gain=125
  Sum1 : Sum  Inputs=|++++
  Sum2 : Sum  Inputs=|++
  Sum3 : Sum  Inputs=|++
  cost of Battery USD : Constant  Value=1130
  cost of Controller USD : Constant  Value=890
  cost of PV module USD : Constant  Value=99
  "cost of electrolysis USD/Kw " : Constant  Value=588.7
  Capital Cost : Outport
  wires:
  Number of PV module/1 -> Sum1/2
  Sum1/1 -> Sum3/2, Gain6/1
  "cost of electrolysis USD/Kw "/1 -> Capacity of electrolysis/1
  Capacity of electrolysis/1 -> Sum2/2, Gain4/1  "Cost of electrolysis"
  cost of Controller USD/1 -> Number of Controll/1
  cost of PV module USD/1 -> Number of PV module/1
  cost of Battery USD/1 -> "Number of battery "/1
  "Number of battery "/1 -> Sum1/3
  Gain6/1 -> Sum3/1  "cost of supplement"
  Gain4/1 -> Sum2/1  "Balance of plant (BOP)"
  Sum2/1 -> Sum1/1  "total cost of Electroysis plant"
  Sum3/1 -> Capital Cost/1  "Capital Cost"
  Number of Controll/1 -> Sum1/4

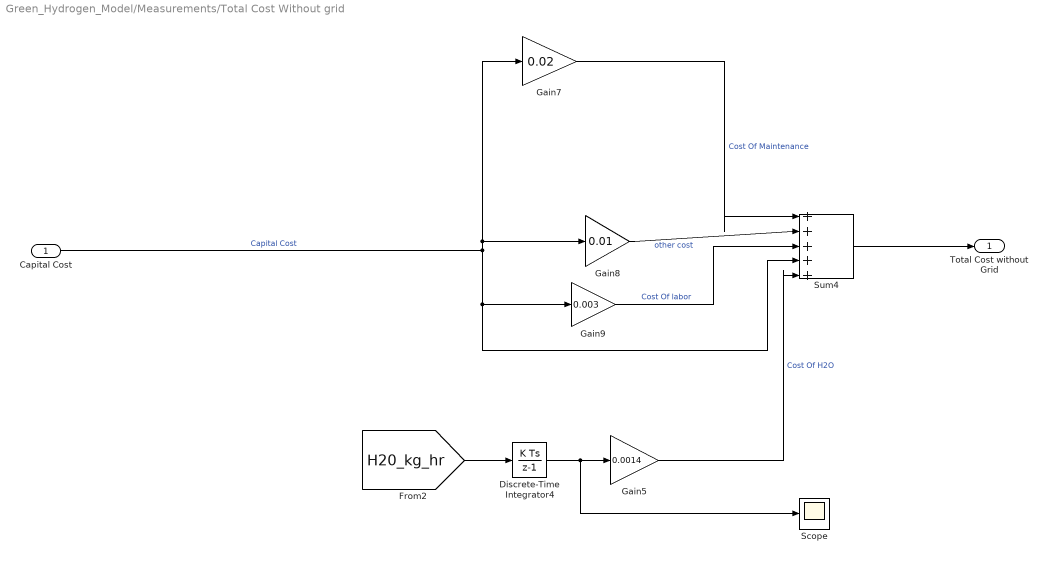
== system Green_Hydrogen_Model/Measurements/Total Cost Without grid ==
  Capital Cost : Inport
  Discrete-Time Integrator4 : DiscreteIntegrator  gainval=1/3600  SampleTime=-1  ICPrevOutput=DiscIntNeverNeededParam  ICPrevScaledInput=DiscIntNeverNeededParam
  Gain5 : Gain  Gain=0.0014
  Gain7 : Gain  Gain=0.02
  Gain8 : Gain  Gain=0.01
  Gain9 : Gain  Gain=0.003
  Scope : Scope
      settings: ActiveDisplayYMinimum=-1.19032063007E+6  ActiveDisplayYMaximum=1.071288567062E+7  DataLoggingVariableName=H2O
  Sum4 : Sum  Inputs=|+++++
  Total Cost without Grid : Outport
  wires:
  Discrete-Time Integrator4/1 -> Scope/1, Gain5/1
  Capital Cost/1 -> Gain7/1, Gain8/1, Gain9/1, Sum4/4  "Capital Cost"
  Gain5/1 -> Sum4/5  "Cost Of H2O"
  Gain8/1 -> Sum4/2  "other cost"
  Gain9/1 -> Sum4/3  "Cost Of labor"
  Gain7/1 -> Sum4/1  "Cost Of Maintenance"
  [H20_kg_hr] -> Discrete-Time Integrator4/1
  Sum4/1 -> Total Cost without Grid/1

== system Green_Hydrogen_Model/Solar Array (ROM)/Buck//Boost ==
  Average-Value DC-DC Converter : ee_lib/Semiconductors & Converters/Converters/Average-Value DC-DC Converter  implementation_option=ee.enum.converters.implementation.behavioral  converter_type=ee.enum.converters.dcdctype.buckboost  control_option=ee.enum.converters.controlinput.dutycycle  efficiency_option=ee.enum.converters.efficiency.constant  efficiency_fixed=95  i_vec=[0, 2, 5] A  efficiency_vec=[90, 95, 98]  Lf=1e-6 H  Rl=0 Ohm  Cf=1e-7 F  Rc=1e-6 Ohm  iL_specify=off  iL_priority=High  iL=0 A  iL_nominal_specify=off  iL_nominal_value=1  iL_nominal_unit=A  vc_specify=off  vc_priority=High  vc=0 V  vc_nominal_specify=off  vc_nominal_value=1  vc_nominal_unit=V
  1+ : PMIOPort  Side=Left
  1- : PMIOPort  Port=2  Side=Left
  DutyCycle : PMIOPort  Port=3  Side=Left
  2+ : PMIOPort  Port=4  Side=Right
  2- : PMIOPort  Port=5  Side=Right
  connections:
  DutyCycle/RConn1 -- Average-Value DC-DC Converter/LConn1
  Average-Value DC-DC Converter/LConn2 -- 1+/RConn1
  1-/RConn1 -- Average-Value DC-DC Converter/LConn3
  Average-Value DC-DC Converter/RConn2 -- 2-/RConn1
  Average-Value DC-DC Converter/RConn1 -- 2+/RConn1

== system Green_Hydrogen_Model/Solar Array (ROM)/Sensing Current ==
  Current Sensor : fl_lib/Electrical/Electrical Sensors/Current Sensor
  PS-Simulink/I : nesl_utility/PS-Simulink Converter  PhysicalDomain=network_engine_domain  SubClassName=ps_output  LeftPortType=input  RightPortType=output  PseudoPeriodic=off  Frequencies=[]  VectorFormat=1-D array  Unit=1  AffineConversion=off
  + : PMIOPort  Side=Left
  - : PMIOPort  Port=2  Side=Right
  tag scope: Isolar=global
  wires:
  PS-Simulink/I/1 -> [Isolar]
  connections:
  Current Sensor/RConn1 -- PS-Simulink/I/LConn1
  Current Sensor/LConn1 -- +/RConn1
  -/RConn1 -- Current Sensor/RConn2

== system Green_Hydrogen_Model/Solar Array (ROM)/sensing voltage ==
  PS-Simulink Converter : nesl_utility/PS-Simulink Converter  PhysicalDomain=network_engine_domain  SubClassName=ps_output  LeftPortType=input  RightPortType=output  PseudoPeriodic=off  Frequencies=[]  VectorFormat=1-D array  Unit=inherit  AffineConversion=off
  Voltage Sensor : fl_lib/Electrical/Electrical Sensors/Voltage Sensor
  + : PMIOPort  Side=Left
  - : PMIOPort  Port=2  Side=Right
  tag scope: Vsolar=global
  wires:
  PS-Simulink Converter/1 -> [Vsolar]
  connections:
  Voltage Sensor/RConn1 -- PS-Simulink Converter/LConn1
  Voltage Sensor/RConn2 -- -/RConn1
  Voltage Sensor/LConn1 -- +/RConn1
